simulink model "PID_Mov"  (R2026b)
settings: Solver=VariableStepAuto
values from neighbouring files (symbols this model uses):
  Kd_mov = wn_mov * (2*zeta_mov + 1) * J_eq    (= 0.0569305555556)    [coeficientes.m]
  Ki_mov = wn_mov^3 * J_eq    (= 14574.2222222)    [coeficientes.m]
  Kp_mov = wn_mov^2 * (2*zeta_mov + 1) * J_eq    (= 45.5444444444)    [coeficientes.m]
settings Model: Creator=admin  LastModifiedBy=fedeb

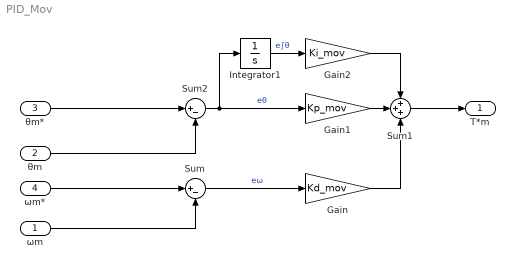
== system PID_Mov ==
  ωm : Inport  Unit=rad/s
  θm : Inport  Port=2
  θm* : Inport  Port=3  Unit=rad/s
  ωm* : Inport  Port=4  Unit=rad/s
  Gain : Gain  Gain=Kd_mov
  Gain1 : Gain  Gain=Kp_mov
  Gain2 : Gain  Gain=Ki_mov
  Integrator1 : Integrator
  Sum : Sum  Inputs=|+-
  Sum1 : Sum  Inputs=+++
  Sum2 : Sum  Inputs=|+-
  T*m : Outport
  wires:
  Gain1/1 -> Sum1/2
  Sum1/1 -> T*m/1
  Gain2/1 -> Sum1/1
  Gain/1 -> Sum1/3
  θm*/1 -> Sum2/1
  Sum/1 -> Gain/1  "eω"
  θm/1 -> Sum2/2
  ωm*/1 -> Sum/1
  ωm/1 -> Sum/2
  Integrator1/1 -> Gain2/1  "e∫θ"
  Sum2/1 -> Integrator1/1, Gain1/1  "eθ"
